simulink model "Fault_RLready_AC_Droop_four_Inverters"  (R2025a)
settings: Solver=ode4  StartTime=0.0  StopTime=15  MaxStep=1e-4  RelTol=1e-3
PreLoadFcn:
  | k_couple = 1;
  | k_power  = 0.0001;
  | k_corr   = 5;
InitFcn:
  | K1=1e-4;
libraries: spsThreePhaseSeriesRLCBranchLib x16, slpidlib x16, spsThreePhaseVIMeasurementLib x12, spsFirstOrderFilterLib x8, spsThreePhaseParallelRLCLoadLib x5, spsDCVoltageSourceLib x4, spsUniversalBridgeLib x4, simulink x4, MGLib x4, spsVoltageMeasurementLib x4, spsThreePhaseBreakerLib x1, spspowerguiLib x1
(part 2 of 4)

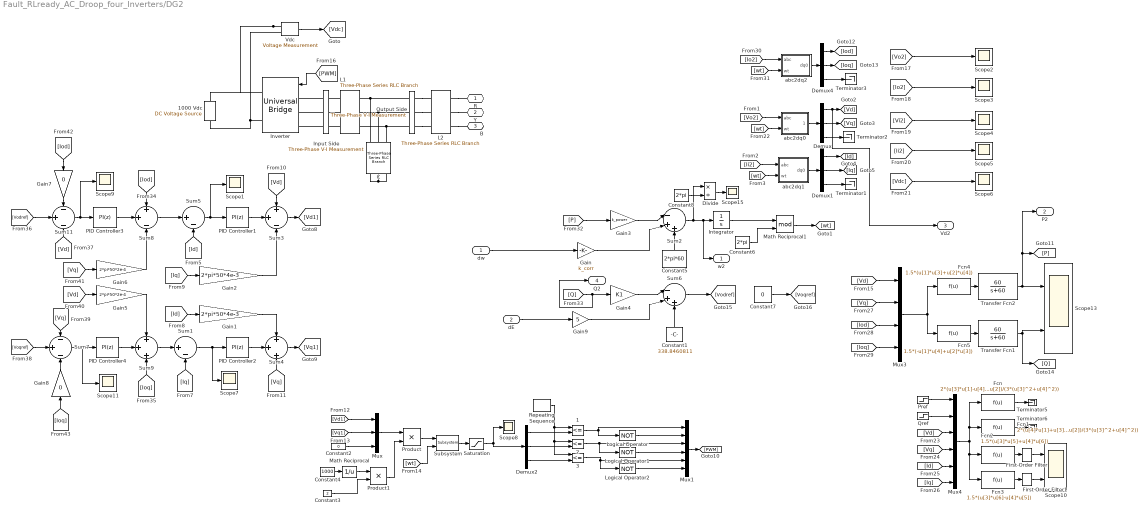
== system Fault_RLready_AC_Droop_four_Inverters/DG2 ==
  dw : Inport
  dE : Inport  Port=2
  1 : RelationalOperator  Operator=<=  OutDataTypeStr=boolean  RndMeth=Simplest  InputSameDT=off
  1000 Vdc : spsDCVoltageSourceLib/DC Voltage Source  Amplitude=1000  Measurements=None
  2 : RelationalOperator  Operator=<=  OutDataTypeStr=boolean  RndMeth=Simplest  InputSameDT=off
  3 : RelationalOperator  Operator=<=  OutDataTypeStr=boolean  RndMeth=Simplest  InputSameDT=off
  C : spsThreePhaseSeriesRLCBranchLib/Three-Phase Series RLC Branch  LConnTagsString=A|B|C  RConnTagsString=A|B|C  BranchType=RC  Resistance=5  Inductance=1e-3  Capacitance=2e-4  Measurements=None
  Constant1 : Constant  Value=338.8460811
  Constant2 : Constant  Value=0
  Constant3 : Constant  Value=2
  Constant4 : Constant  Value=1000
  Constant5 : Constant  Value=2*pi*60
  Constant6 : Constant  Value=2*pi
  Constant7 : Constant  Value=0
  Constant8 : Constant  Value=2*pi
  Demux{,1..2,4} (4 alike) : Demux  Outputs=3
  Divide : Product  Inputs=*/
  Fcn : Fcn  Expr=2*(u[3]*u[1]-u[4]*u[2])/(3*(u[3]^2+u[4]^2))
  Fcn1 : Fcn  Expr=2*(u[4]*u[1]+u[3]*u[2])/(3*(u[3]^2+u[4]^2))
  Fcn2 : Fcn  Expr=1.5*(u[3]*u[5]+u[4]*u[6])
  Fcn3 : Fcn  Expr=1.5*(u[3]*u[6]-u[4]*u[5])
  Fcn4 : Fcn  Expr=1.5*(u[1]*u[3]+u[2]*u[4])
  Fcn5 : Fcn  Expr=1.5*(-u[1]*u[4]+u[2]*u[3])
  First-Order Filter : spsFirstOrderFilterLib/First-Order Filter  FilterType=Lowpass  Tc=0.03  Ts=0  Initialize=on  Vac_Init=[0, 0, 60]  Vdc_Init=0  PlotResponse=off  FreqRange="[0,  200,  1]"
  First-Order Filter1 : spsFirstOrderFilterLib/First-Order Filter  FilterType=Lowpass  Tc=0.03  Ts=0  Initialize=on  Vac_Init=[0, 0, 60]  Vdc_Init=0  PlotResponse=off  FreqRange="[0,  200,  1]"
  Gain : Gain  Gain=k_corr
  Gain1 : Gain  Gain=2*pi*50*4e-3
  Gain2 : Gain  Gain=2*pi*50*4e-3
  Gain3 : Gain  Gain=k_power
  Gain4 : Gain  Gain=K1
  Gain5 : Gain  Gain=2*pi*50*2e-4
  Gain6 : Gain  Gain=2*pi*50*2e-4
  Gain7 : Gain  Gain=0
  Gain8 : Gain  Gain=0
  Gain9 : Gain  Gain=5
  Input Side : spsThreePhaseVIMeasurementLib/Three-Phase V-I Measurement  VoltageMeasurement=phase-to-ground  SetLabelV=on  LabelV=Vi2  Vpu=off  VpuLL=off  CurrentMeasurement=yes  SetLabelI=on  LabelI=Ii2  Ipu=off  Pbase=100e6  Vbase=500e3  OutputType=Complex  PhasorSimulation=off  PSBequivalent=0
  Integrator : Integrator
  Inverter : spsUniversalBridgeLib/Universal Bridge  Arms=3  SnubberResistance=1e5  SnubberCapacitance=inf  Device=Ideal Switches  Ron=1e-3  Lon=0  ForwardVoltages="[  0  0  ]"  ForwardVoltage=0  GTOparameters=[ 10e-6 , 20e-6 ]  IGBTparameters=[ 1e-6 , 2e-6 ]  Measurements=None  Measurements_2=None  converterType=Rectifier
  L1 : spsThreePhaseSeriesRLCBranchLib/Three-Phase Series RLC Branch  LConnTagsString=A|B|C  RConnTagsString=A|B|C  BranchType=RL  Resistance=0.1  Inductance=4e-3  Capacitance=1e-6  Measurements=None
  L2 : spsThreePhaseSeriesRLCBranchLib/Three-Phase Series RLC Branch  LConnTagsString=A|B|C  RConnTagsString=A|B|C  BranchType=RL  Resistance=0.03  Inductance=1e-3  Capacitance=1e-6  Measurements=None
  Logical Operator : Logic  Operator=NOT  IconShape=distinctive  AllPortsSameDT=off  OutDataTypeStr=boolean
  Logical Operator1 : Logic  Operator=NOT  IconShape=distinctive  AllPortsSameDT=off  OutDataTypeStr=boolean
  Logical Operator2 : Logic  Operator=NOT  IconShape=distinctive  AllPortsSameDT=off  OutDataTypeStr=boolean
  Math Reciprocal : Math  Operator=reciprocal  SignedPower=on
  Math Reciprocal1 : Math  Operator=mod  SignedPower=on
  Mux : Mux  Inputs=3
  Mux1 : Mux  Inputs=6
  Mux3 : Mux
  Mux4 : Mux  Inputs=6
  Output Side : spsThreePhaseVIMeasurementLib/Three-Phase V-I Measurement  VoltageMeasurement=phase-to-ground  SetLabelV=on  LabelV=Vo2  Vpu=off  VpuLL=off  CurrentMeasurement=yes  SetLabelI=on  LabelI=Io2  Ipu=off  Pbase=100e6  Vbase=500e3  OutputType=Complex  PhasorSimulation=off  PSBequivalent=0
  PID Controller1 : slpidlib/PID Controller  Controller=PI  Form=Parallel  TimeDomain=Discrete-time  UseExternalTs=off  SampleTime=-1  IntegratorMethod=Forward Euler  FilterMethod=Forward Euler  ControllerParametersSource=internal  P=4e-3/1e-4  I=0.1/1e-4  UseKiTs=off  D=0  UseExternalDerivativeSource=off  N=100  UseFilter=on  TunerSelectOption=Transfer Function Based (PID Tuner App)  InitialConditionSource=internal  InitialConditionForIntegrator=0  InitialConditionForFilter=0  DifferentiatorICPrevScaledInput=0  ExternalReset=none  TrackingMode=off  Kt=1  LimitOutput=off  SatLimitsSource=internal  UpperSaturationLimit=inf  LowerSaturationLimit=-inf  LinearizeAsGain=on  AntiWindupMode=none  Kb=1  LimitIntegrator=off  UpperIntegratorSaturationLimit=inf  LowerIntegratorSaturationLimit=-inf  POutMin=[]  POutMax=[]  IOutMin=[]  IOutMax=[]  DOutMin=[]  DOutMax=[]  NOutMin=[]  NOutMax=[]  SumOutMin=[]  SumOutMax=[]  SaturationOutMin=[]  SaturationOutMax=[]  PParamMin=[]  PParamMax=[]  IParamMin=[]  IParamMax=[]  DParamMin=[]  DParamMax=[]  NParamMin=[]  NParamMax=[]  KbParamMin=[]  KbParamMax=[]  KtParamMin=[]  KtParamMax=[]  KbOutMin=[]  KbOutMax=[]  KtOutMin=[]  KtOutMax=[]  IntegratorOutMin=[]  IntegratorOutMax=[]  FilterOutMin=[]  FilterOutMax=[]  SumI1OutMin=[]  SumI1OutMax=[]  SumI2OutMin=[]  SumI2OutMax=[]  SumI3OutMin=[]  SumI3OutMax=[]  SumI4OutMin=[]  SumI4OutMax=[]  SumDOutMin=[]  SumDOutMax=[]  DifferentiatorOutMin=[]  DifferentiatorOutMax=[]  FilterDiffOutCoefMin=[]  FilterDiffOutCoefMax=[]  ReciprocalOutMin=[]  ReciprocalOutMax=[]  SumDenOutMin=[]  SumDenOutMax=[]  SumNumOutMin=[]  SumNumOutMax=[]  DivideOutMin=[]  DivideOutMax=[]  UdiffTsProdOutMin=[]  UdiffTsProdOutMax=[]  NTsProdOutMin=[]  NTsProdOutMax=[]  UintegralTsProdOutMin=[]  UintegralTsProdOutMax=[]  UngainTsProdOutMin=[]  UngainTsProdOutMax=[]  ClampingZeroOutDataTypeStr=Inherit: Inherit via back propagation  ClampingZeroOutMin=[]  ClampingZeroOutMax=[]  FilterDenConstantOutDataTypeStr=Inherit: Inherit via back propagation  FilterDenConstantOutMin=[]  FilterDenConstantOutMax=[]  PCopyOutDataTypeStr=Inherit: Inherit via back propagation  PCopyOutMin=[]  PCopyOutMax=[]  NCopyOutDataTypeStr=Inherit: Inherit via back propagation  NCopyOutMin=[]  NCopyOutMax=[]  IntegratorContinuousStateAttributes=''  IntegratorStateMustResolveToSignalObject=off  IntegratorRTWStateStorageClass=Auto  FilterContinuousStateAttributes=''  FilterStateMustResolveToSignalObject=off  FilterRTWStateStorageClass=Auto  ParallelPVariant=InternalParameters  IdealPVariant=Disabled  IVariant=InternalParameters  DVariant=Disabled  IntegratorVariant=Discrete  SatVariant=Disabled  AWVariant=Passthrough  PCopyVariant=Disabled  TRVariant=Disabled  FdbkBlocksVariant=Forward  IdealPFdbkVariant=Disabled  SatFdbkVariant=Disabled  DerivativeFilterVariant=Disabled  NVariant=Disabled  NCopyVariant=Disabled_SignalSpec  FilterICVariant=Disabled  IntegratorICVariant=InternalICs  ExternalResetVariant=Disabled  TRSumVariant=Passthrough  SumFdbkVariant=Disabled  SumVariant=Sum_PI  TsampFilterVariant=InternalTs  TsampNgainVariant=Passthrough  TsampIntegralVariant=Disabled_SignalSpec  ExternalSaturationOutDataTypeStr=Inherit: Same as second input  DerivativeSourceVariant=Disabled  PreIntVariant=InternalPreInt
  PID Controller2 : slpidlib/PID Controller  Controller=PI  Form=Parallel  TimeDomain=Discrete-time  UseExternalTs=off  SampleTime=-1  IntegratorMethod=Forward Euler  FilterMethod=Forward Euler  ControllerParametersSource=internal  P=4e-3/1e-4  I=0.1/1e-4  UseKiTs=off  D=0  UseExternalDerivativeSource=off  N=100  UseFilter=on  TunerSelectOption=Transfer Function Based (PID Tuner App)  InitialConditionSource=internal  InitialConditionForIntegrator=0  InitialConditionForFilter=0  DifferentiatorICPrevScaledInput=0  ExternalReset=none  TrackingMode=off  Kt=1  LimitOutput=off  SatLimitsSource=internal  UpperSaturationLimit=inf  LowerSaturationLimit=-inf  LinearizeAsGain=on  AntiWindupMode=none  Kb=1  LimitIntegrator=off  UpperIntegratorSaturationLimit=inf  LowerIntegratorSaturationLimit=-inf  POutMin=[]  POutMax=[]  IOutMin=[]  IOutMax=[]  DOutMin=[]  DOutMax=[]  NOutMin=[]  NOutMax=[]  SumOutMin=[]  SumOutMax=[]  SaturationOutMin=[]  SaturationOutMax=[]  PParamMin=[]  PParamMax=[]  IParamMin=[]  IParamMax=[]  DParamMin=[]  DParamMax=[]  NParamMin=[]  NParamMax=[]  KbParamMin=[]  KbParamMax=[]  KtParamMin=[]  KtParamMax=[]  KbOutMin=[]  KbOutMax=[]  KtOutMin=[]  KtOutMax=[]  IntegratorOutMin=[]  IntegratorOutMax=[]  FilterOutMin=[]  FilterOutMax=[]  SumI1OutMin=[]  SumI1OutMax=[]  SumI2OutMin=[]  SumI2OutMax=[]  SumI3OutMin=[]  SumI3OutMax=[]  SumI4OutMin=[]  SumI4OutMax=[]  SumDOutMin=[]  SumDOutMax=[]  DifferentiatorOutMin=[]  DifferentiatorOutMax=[]  FilterDiffOutCoefMin=[]  FilterDiffOutCoefMax=[]  ReciprocalOutMin=[]  ReciprocalOutMax=[]  SumDenOutMin=[]  SumDenOutMax=[]  SumNumOutMin=[]  SumNumOutMax=[]  DivideOutMin=[]  DivideOutMax=[]  UdiffTsProdOutMin=[]  UdiffTsProdOutMax=[]  NTsProdOutMin=[]  NTsProdOutMax=[]  UintegralTsProdOutMin=[]  UintegralTsProdOutMax=[]  UngainTsProdOutMin=[]  UngainTsProdOutMax=[]  ClampingZeroOutDataTypeStr=Inherit: Inherit via back propagation  ClampingZeroOutMin=[]  ClampingZeroOutMax=[]  FilterDenConstantOutDataTypeStr=Inherit: Inherit via back propagation  FilterDenConstantOutMin=[]  FilterDenConstantOutMax=[]  PCopyOutDataTypeStr=Inherit: Inherit via back propagation  PCopyOutMin=[]  PCopyOutMax=[]  NCopyOutDataTypeStr=Inherit: Inherit via back propagation  NCopyOutMin=[]  NCopyOutMax=[]  IntegratorContinuousStateAttributes=''  IntegratorStateMustResolveToSignalObject=off  IntegratorRTWStateStorageClass=Auto  FilterContinuousStateAttributes=''  FilterStateMustResolveToSignalObject=off  FilterRTWStateStorageClass=Auto  ParallelPVariant=InternalParameters  IdealPVariant=Disabled  IVariant=InternalParameters  DVariant=Disabled  IntegratorVariant=Discrete  SatVariant=Disabled  AWVariant=Passthrough  PCopyVariant=Disabled  TRVariant=Disabled  FdbkBlocksVariant=Forward  IdealPFdbkVariant=Disabled  SatFdbkVariant=Disabled  DerivativeFilterVariant=Disabled  NVariant=Disabled  NCopyVariant=Disabled_SignalSpec  FilterICVariant=Disabled  IntegratorICVariant=InternalICs  ExternalResetVariant=Disabled  TRSumVariant=Passthrough  SumFdbkVariant=Disabled  SumVariant=Sum_PI  TsampFilterVariant=InternalTs  TsampNgainVariant=Passthrough  TsampIntegralVariant=Disabled_SignalSpec  ExternalSaturationOutDataTypeStr=Inherit: Same as second input  DerivativeSourceVariant=Disabled  PreIntVariant=InternalPreInt
  PID Controller3 : slpidlib/PID Controller  Controller=PI  Form=Parallel  TimeDomain=Discrete-time  UseExternalTs=off  SampleTime=-1  IntegratorMethod=Forward Euler  FilterMethod=Forward Euler  ControllerParametersSource=internal  P=2e-4/1e-3  I=5/1e-3  UseKiTs=off  D=0  UseExternalDerivativeSource=off  N=100  UseFilter=on  TunerSelectOption=Transfer Function Based (PID Tuner App)  InitialConditionSource=internal  InitialConditionForIntegrator=0  InitialConditionForFilter=0  DifferentiatorICPrevScaledInput=0  ExternalReset=none  TrackingMode=off  Kt=1  LimitOutput=off  SatLimitsSource=internal  UpperSaturationLimit=inf  LowerSaturationLimit=-inf  LinearizeAsGain=on  AntiWindupMode=none  Kb=1  LimitIntegrator=off  UpperIntegratorSaturationLimit=inf  LowerIntegratorSaturationLimit=-inf  POutMin=[]  POutMax=[]  IOutMin=[]  IOutMax=[]  DOutMin=[]  DOutMax=[]  NOutMin=[]  NOutMax=[]  SumOutMin=[]  SumOutMax=[]  SaturationOutMin=[]  SaturationOutMax=[]  PParamMin=[]  PParamMax=[]  IParamMin=[]  IParamMax=[]  DParamMin=[]  DParamMax=[]  NParamMin=[]  NParamMax=[]  KbParamMin=[]  KbParamMax=[]  KtParamMin=[]  KtParamMax=[]  KbOutMin=[]  KbOutMax=[]  KtOutMin=[]  KtOutMax=[]  IntegratorOutMin=[]  IntegratorOutMax=[]  FilterOutMin=[]  FilterOutMax=[]  SumI1OutMin=[]  SumI1OutMax=[]  SumI2OutMin=[]  SumI2OutMax=[]  SumI3OutMin=[]  SumI3OutMax=[]  SumI4OutMin=[]  SumI4OutMax=[]  SumDOutMin=[]  SumDOutMax=[]  DifferentiatorOutMin=[]  DifferentiatorOutMax=[]  FilterDiffOutCoefMin=[]  FilterDiffOutCoefMax=[]  ReciprocalOutMin=[]  ReciprocalOutMax=[]  SumDenOutMin=[]  SumDenOutMax=[]  SumNumOutMin=[]  SumNumOutMax=[]  DivideOutMin=[]  DivideOutMax=[]  UdiffTsProdOutMin=[]  UdiffTsProdOutMax=[]  NTsProdOutMin=[]  NTsProdOutMax=[]  UintegralTsProdOutMin=[]  UintegralTsProdOutMax=[]  UngainTsProdOutMin=[]  UngainTsProdOutMax=[]  ClampingZeroOutDataTypeStr=Inherit: Inherit via back propagation  ClampingZeroOutMin=[]  ClampingZeroOutMax=[]  FilterDenConstantOutDataTypeStr=Inherit: Inherit via back propagation  FilterDenConstantOutMin=[]  FilterDenConstantOutMax=[]  PCopyOutDataTypeStr=Inherit: Inherit via back propagation  PCopyOutMin=[]  PCopyOutMax=[]  NCopyOutDataTypeStr=Inherit: Inherit via back propagation  NCopyOutMin=[]  NCopyOutMax=[]  IntegratorContinuousStateAttributes=''  IntegratorStateMustResolveToSignalObject=off  IntegratorRTWStateStorageClass=Auto  FilterContinuousStateAttributes=''  FilterStateMustResolveToSignalObject=off  FilterRTWStateStorageClass=Auto  ParallelPVariant=InternalParameters  IdealPVariant=Disabled  IVariant=InternalParameters  DVariant=Disabled  IntegratorVariant=Discrete  SatVariant=Disabled  AWVariant=Passthrough  PCopyVariant=Disabled  TRVariant=Disabled  FdbkBlocksVariant=Forward  IdealPFdbkVariant=Disabled  SatFdbkVariant=Disabled  DerivativeFilterVariant=Disabled  NVariant=Disabled  NCopyVariant=Disabled_SignalSpec  FilterICVariant=Disabled  IntegratorICVariant=InternalICs  ExternalResetVariant=Disabled  TRSumVariant=Passthrough  SumFdbkVariant=Disabled  SumVariant=Sum_PI  TsampFilterVariant=InternalTs  TsampNgainVariant=Passthrough  TsampIntegralVariant=Disabled_SignalSpec  ExternalSaturationOutDataTypeStr=Inherit: Same as second input  DerivativeSourceVariant=Disabled  PreIntVariant=InternalPreInt
  PID Controller4 : slpidlib/PID Controller  Controller=PI  Form=Parallel  TimeDomain=Discrete-time  UseExternalTs=off  SampleTime=-1  IntegratorMethod=Forward Euler  FilterMethod=Forward Euler  ControllerParametersSource=internal  P=2e-4/1e-3  I=5/1e-3  UseKiTs=off  D=0  UseExternalDerivativeSource=off  N=100  UseFilter=on  TunerSelectOption=Transfer Function Based (PID Tuner App)  InitialConditionSource=internal  InitialConditionForIntegrator=0  InitialConditionForFilter=0  DifferentiatorICPrevScaledInput=0  ExternalReset=none  TrackingMode=off  Kt=1  LimitOutput=off  SatLimitsSource=internal  UpperSaturationLimit=inf  LowerSaturationLimit=-inf  LinearizeAsGain=on  AntiWindupMode=none  Kb=1  LimitIntegrator=off  UpperIntegratorSaturationLimit=inf  LowerIntegratorSaturationLimit=-inf  POutMin=[]  POutMax=[]  IOutMin=[]  IOutMax=[]  DOutMin=[]  DOutMax=[]  NOutMin=[]  NOutMax=[]  SumOutMin=[]  SumOutMax=[]  SaturationOutMin=[]  SaturationOutMax=[]  PParamMin=[]  PParamMax=[]  IParamMin=[]  IParamMax=[]  DParamMin=[]  DParamMax=[]  NParamMin=[]  NParamMax=[]  KbParamMin=[]  KbParamMax=[]  KtParamMin=[]  KtParamMax=[]  KbOutMin=[]  KbOutMax=[]  KtOutMin=[]  KtOutMax=[]  IntegratorOutMin=[]  IntegratorOutMax=[]  FilterOutMin=[]  FilterOutMax=[]  SumI1OutMin=[]  SumI1OutMax=[]  SumI2OutMin=[]  SumI2OutMax=[]  SumI3OutMin=[]  SumI3OutMax=[]  SumI4OutMin=[]  SumI4OutMax=[]  SumDOutMin=[]  SumDOutMax=[]  DifferentiatorOutMin=[]  DifferentiatorOutMax=[]  FilterDiffOutCoefMin=[]  FilterDiffOutCoefMax=[]  ReciprocalOutMin=[]  ReciprocalOutMax=[]  SumDenOutMin=[]  SumDenOutMax=[]  SumNumOutMin=[]  SumNumOutMax=[]  DivideOutMin=[]  DivideOutMax=[]  UdiffTsProdOutMin=[]  UdiffTsProdOutMax=[]  NTsProdOutMin=[]  NTsProdOutMax=[]  UintegralTsProdOutMin=[]  UintegralTsProdOutMax=[]  UngainTsProdOutMin=[]  UngainTsProdOutMax=[]  ClampingZeroOutDataTypeStr=Inherit: Inherit via back propagation  ClampingZeroOutMin=[]  ClampingZeroOutMax=[]  FilterDenConstantOutDataTypeStr=Inherit: Inherit via back propagation  FilterDenConstantOutMin=[]  FilterDenConstantOutMax=[]  PCopyOutDataTypeStr=Inherit: Inherit via back propagation  PCopyOutMin=[]  PCopyOutMax=[]  NCopyOutDataTypeStr=Inherit: Inherit via back propagation  NCopyOutMin=[]  NCopyOutMax=[]  IntegratorContinuousStateAttributes=''  IntegratorStateMustResolveToSignalObject=off  IntegratorRTWStateStorageClass=Auto  FilterContinuousStateAttributes=''  FilterStateMustResolveToSignalObject=off  FilterRTWStateStorageClass=Auto  ParallelPVariant=InternalParameters  IdealPVariant=Disabled  IVariant=InternalParameters  DVariant=Disabled  IntegratorVariant=Discrete  SatVariant=Disabled  AWVariant=Passthrough  PCopyVariant=Disabled  TRVariant=Disabled  FdbkBlocksVariant=Forward  IdealPFdbkVariant=Disabled  SatFdbkVariant=Disabled  DerivativeFilterVariant=Disabled  NVariant=Disabled  NCopyVariant=Disabled_SignalSpec  FilterICVariant=Disabled  IntegratorICVariant=InternalICs  ExternalResetVariant=Disabled  TRSumVariant=Passthrough  SumFdbkVariant=Disabled  SumVariant=Sum_PI  TsampFilterVariant=InternalTs  TsampNgainVariant=Passthrough  TsampIntegralVariant=Disabled_SignalSpec  ExternalSaturationOutDataTypeStr=Inherit: Same as second input  DerivativeSourceVariant=Disabled  PreIntVariant=InternalPreInt
  Pref : Step  Time=10  Before=10000  After=15000  SampleTime=0
  Product : Product
  Product1 : Product
  Qref : Step  Time=10  Before=54.1077  After=400  SampleTime=0
  Repeating Sequence : simulink/Sources/Repeating Sequence  rep_seq_t=[0 0.25 .5 0.75 1]/10000  rep_seq_y=[0 +1 0 -1 0]
  Saturation : Saturate  UpperLimit=1  LowerLimit=-1
  Scope{1..9,11,15} (11 alike) : Scope
      Scope1 settings: ActiveDisplayYMinimum=-49.45655  ActiveDisplayYMaximum=291.1825
      Scope11 settings: ActiveDisplayYMinimum=-70.8299  ActiveDisplayYMaximum=49.76982
      Scope15 settings: ActiveDisplayYMinimum=59.272227157969354  ActiveDisplayYMaximum=60.080912604983666
      Scope2 settings: ActiveDisplayYMinimum=-481.79005  ActiveDisplayYMaximum=381.24377  DataLoggingVariableName=ScopeData5
      Scope3 settings: ActiveDisplayYMinimum=-55.99784  ActiveDisplayYMaximum=55.98753  DataLoggingVariableName=ScopeData6
      Scope4 settings: ActiveDisplayYMinimum=-702.35556  ActiveDisplayYMaximum=784.25935  DataLoggingVariableName=ScopeData7
      Scope5 settings: ActiveDisplayYMinimum=-20.37356  ActiveDisplayYMaximum=18.38892  DataLoggingVariableName=ScopeData8
      Scope6 settings: ActiveDisplayYMinimum=600  ActiveDisplayYMaximum=800  DataLoggingVariableName=ScopeData9
      Scope7 settings: ActiveDisplayYMinimum=-104.85977  ActiveDisplayYMaximum=99.61637  DataLoggingVariableName=ScopeData2
      Scope8 settings: ActiveDisplayYMinimum=0.61458  ActiveDisplayYMaximum=0.66041  DataLoggingVariableName=ScopeData3
      Scope9 settings: ActiveDisplayYMinimum=-392.5882  ActiveDisplayYMaximum=763.99218  DataLoggingVariableName=ScopeData2
  Scope10 : Scope  NumInputPorts=2
      settings: ActiveDisplayYMinimum=-1742.84392  ActiveDisplayYMaximum=15685.45556  DataLoggingVariableName=ScopeData10
  Scope13 : Scope  NumInputPorts=2
      settings: ActiveDisplayYMinimum=-5370.8227360639794  ActiveDisplayYMaximum=48337.400439217869  DataLoggingVariableName=ScopeData11
  Subsystem : MGLib/Subsystem  Power=Power Variant  dq=q-axis leads d-axis  Alignment=90 deg. behind a-phase axis
  Sum1 : Sum  Inputs=|+-
  Sum11 : Sum  Inputs=-|+|-
  Sum2 : Sum  Inputs=|-++
  Sum3 : Sum  Inputs=+|+|-
  Sum4 : Sum  Inputs=+|+|+
  Sum5 : Sum  Inputs=|+-
  Sum6 : Sum  Inputs=|-++
  Sum7 : Sum  Inputs=-|+|-
  Sum8 : Sum  Inputs=+|+|-
  Sum9 : Sum  Inputs=+|+|+
  Terminator{1..3,5..6} (5 alike) : Terminator
  Transfer Fcn1 : TransferFcn  Numerator=60  Denominator=[1 60]
  Transfer Fcn2 : TransferFcn  Numerator=60  Denominator=[1 60]
  Vdc : spsVoltageMeasurementLib/Voltage Measurement  PhasorSimulation=off  OutputType=Complex  PSBequivalent=0
  abc2dq0 : Subsystem  mask(abc to dq0 Transformation){Power=Power Variant, dq=q-axis leads d-axis, Alignment=90 deg. behind a-phase axis}
      mask prompts: Power "Power Variant/Invariant"; dq "d-q Axes Arrangement"; Alignment "Rotating frame alignment at wt=0"
      mask init: same as Fault_RLready_AC_Droop_four_Inverters/DG1/abc2dq0
      mask TypeOptions Power: Power Variant | Power Invariant
      mask TypeOptions dq: q-axis leads d-axis | q-axis lags d-axis
      mask TypeOptions Alignment: Along a-phase axis | 90 deg. behind a-phase axis
      mask Display:
      | plot([0 1], [0,1])
      | port_label('input', 1, 'abc')
      | port_label('input', 2, 'wt')
      | port_label('output', 1, 'dq0')
  abc2dq1 : Subsystem  mask(abc to dq0 Transformation){Power=Power Variant, dq=q-axis leads d-axis, Alignment=90 deg. behind a-phase axis}
      mask prompts: Power "Power Variant/Invariant"; dq "d-q Axes Arrangement"; Alignment "Rotating frame alignment at wt=0"
      mask init: same as Fault_RLready_AC_Droop_four_Inverters/DG1/abc2dq0
      mask TypeOptions Power: Power Variant | Power Invariant
      mask TypeOptions dq: q-axis leads d-axis | q-axis lags d-axis
      mask TypeOptions Alignment: Along a-phase axis | 90 deg. behind a-phase axis
      mask Display:
      | plot([0 1], [0,1])
      | port_label('input', 1, 'abc')
      | port_label('input', 2, 'wt')
      | port_label('output', 1, 'dq0')
  abc2dq2 : Subsystem  mask(abc to dq0 Transformation){Power=Power Variant, dq=q-axis leads d-axis, Alignment=90 deg. behind a-phase axis}
      mask prompts: Power "Power Variant/Invariant"; dq "d-q Axes Arrangement"; Alignment "Rotating frame alignment at wt=0"
      mask init: same as Fault_RLready_AC_Droop_four_Inverters/DG1/abc2dq0
      mask TypeOptions Power: Power Variant | Power Invariant
      mask TypeOptions dq: q-axis leads d-axis | q-axis lags d-axis
      mask TypeOptions Alignment: Along a-phase axis | 90 deg. behind a-phase axis
      mask Display:
      | plot([0 1], [0,1])
      | port_label('input', 1, 'abc')
      | port_label('input', 2, 'wt')
      | port_label('output', 1, 'dq0')
  R : PMIOPort  Side=Right
  Y : PMIOPort  Port=2  Side=Right
  B : PMIOPort  Port=3  Side=Right
  w2 : Outport  VectorParamsAs1DForOutWhenUnconnected=off
  P2 : Outport  Port=2  VectorParamsAs1DForOutWhenUnconnected=off
  Vd2 : Outport  Port=3  VectorParamsAs1DForOutWhenUnconnected=off
  Q2 : Outport  Port=4  VectorParamsAs1DForOutWhenUnconnected=off
  wires:
  Constant7/1 -> [Voqref]
  Sum6/1 -> [Vodref]
  Math Reciprocal1/1 -> [wt]
  Constant6/1 -> Math Reciprocal1/2
  Integrator/1 -> Math Reciprocal1/1
  Gain4/1 -> Sum6/1
  [Q] -> Q2/1, Gain4/1
  Gain3/1 -> Sum2/1
  [P] -> Gain3/1
  Sum8/1 -> Sum5/1
  [wt] -> abc2dq2/2(wt)
  [wt] -> abc2dq0/2(wt)
  [wt] -> abc2dq1/2(wt)
  [PWM] -> Inverter/1
  abc2dq1/1(dq0) -> Demux1/1
  Demux/1 -> Vd2/1, [Vd]
  [Ii2] -> Scope5/1
  [Io2] -> Scope3/1
  [Vo2] -> abc2dq0/1(abc)
  [Ii2] -> abc2dq1/1(abc)
  Demux1/2 -> [Iq]
  abc2dq2/1(dq0) -> Demux4/1
  [Vi2] -> Scope4/1
  [Vdc] -> Scope6/1
  [Io2] -> abc2dq2/1(abc)
  Demux1/1 -> [Id]
  Demux/3 -> Terminator2/1
  [Vo2] -> Scope2/1
  Demux4/2 -> [Ioq]
  abc2dq0/1(dq0) -> Demux/1
  Demux4/1 -> [Iod]
  Demux4/3 -> Terminator3/1
  Demux/2 -> [Vq]
  Demux1/3 -> Terminator1/1
  PID Controller2/1 -> Sum4/2
  Gain2/1 -> Sum3/3
  Constant4/1 -> Math Reciprocal/1
  Sum1/1 -> PID Controller2/1, Scope7/1
  [Id] -> Sum5/2
  Product/1 -> Subsystem/1
  Product1/1 -> Product/2
  2/1 -> Mux1/3, Logical Operator1/1
  [Vd1] -> Mux/1
  Logical Operator/1 -> Mux1/2
  Gain1/1 -> Sum4/1
  Constant2/1 -> Mux/3
  [Vq1] -> Mux/2
  Sum9/1 -> Sum1/1
  [Vd] -> Sum3/1
  Subsystem/1 -> Saturation/1
  [wt] -> Subsystem/2
  Constant3/1 -> Product1/2
  3/1 -> Mux1/5, Logical Operator2/1
  Math Reciprocal/1 -> Product1/1
  Logical Operator1/1 -> Mux1/4
  PID Controller1/1 -> Sum3/2
  [Iq] -> Sum1/2
  Sum5/1 -> PID Controller1/1, Scope1/1
  Logical Operator2/1 -> Mux1/6
  Sum4/1 -> [Vq1]
  Mux/1 -> Product/1
  Demux2/3 -> 3/2
  Sum3/1 -> [Vd1]
  [Id] -> Gain1/1
  [Iq] -> Gain2/1
  Mux1/1 -> [PWM]
  [Vq] -> Sum4/3
  Saturation/1 -> Scope8/1, Demux2/1
  Repeating Sequence/1 -> 1/1, 2/1, 3/1
  Demux2/2 -> 2/2
  Demux2/1 -> 1/2
  1/1 -> Logical Operator/1, Mux1/1
  Transfer Fcn1/1 -> [Q], Scope13/2
  Fcn3/1 -> First-Order Filter1/1
  Qref/1 -> Mux4/2
  First-Order Filter1/1 -> Scope10/2
  Fcn5/1 -> Transfer Fcn1/1
  [Ioq] -> Mux3/4
  Fcn4/1 -> Transfer Fcn2/1
  First-Order Filter/1 -> Scope10/1
  [Vd] -> Mux4/3
  Fcn2/1 -> First-Order Filter/1
  Mux4/1 -> Fcn/1, Fcn1/1, Fcn3/1, Fcn2/1
  [Id] -> Mux4/5
  Pref/1 -> Mux4/1
  Transfer Fcn2/1 -> Scope13/1, P2/1, [P]
  Fcn1/1 -> Terminator6/1
  [Iq] -> Mux4/6
  [Vq] -> Mux4/4
  [Vq] -> Mux3/2
  [Vd] -> Mux3/1
  Mux3/1 -> Fcn4/1, Fcn5/1
  [Iod] -> Mux3/3
  Fcn/1 -> Terminator5/1
  Vdc/1 -> [Vdc]
  Sum2/1 -> Divide/1, w2/1, Integrator/1
  Divide/1 -> Scope15/1
  Constant8/1 -> Divide/2
  [Ioq] -> Gain8/1
  Gain8/1 -> Sum7/3
  Sum11/1 -> PID Controller3/1, Scope9/1
  [Vodref] -> Sum11/2
  [Vd] -> Gain5/1
  [Vq] -> Sum7/1
  [Vq] -> Gain6/1
  [Iod] -> Sum8/1
  [Vd] -> Sum11/3
  [Ioq] -> Sum9/3
  Sum7/1 -> PID Controller4/1, Scope11/1
  Gain5/1 -> Sum9/1
  Gain6/1 -> Sum8/3
  [Voqref] -> Sum7/2
  [Iod] -> Gain7/1
  Gain7/1 -> Sum11/1
  PID Controller3/1 -> Sum8/2
  PID Controller4/1 -> Sum9/2
  Constant5/1 -> Sum2/3
  Gain/1 -> Sum2/2
  dw/1 -> Gain/1
  Constant1/1 -> Sum6/3
  dE/1 -> Gain9/1
  Gain9/1 -> Sum6/2
  connections:
  C/RConn2 -- C/RConn3 -- C/RConn1
  Input Side/LConn2 -- Inverter/LConn2
  L1/LConn3 -- Input Side/RConn3
  Input Side/LConn3 -- Inverter/LConn3
  Input Side/LConn1 -- Inverter/LConn1
  1000 Vdc/LConn1 -- Vdc/LConn2 -- Inverter/RConn2
  L1/LConn1 -- Input Side/RConn1
  L1/LConn2 -- Input Side/RConn2
  Vdc/LConn1 -- 1000 Vdc/RConn1 -- Inverter/RConn1
  C/LConn2 -- Output Side/LConn2 -- L1/RConn2
  C/LConn3 -- L1/RConn3 -- Output Side/LConn3
  C/LConn1 -- Output Side/LConn1 -- L1/RConn1
  L2/RConn1 -- R/RConn1
  L2/RConn2 -- Y/RConn1
  L2/RConn3 -- B/RConn1
  Output Side/RConn1 -- L2/LConn1
  Output Side/RConn2 -- L2/LConn2
  Output Side/RConn3 -- L2/LConn3
